simulink model "non_ACC"  (R2021b)
settings: Solver=ode5  StartTime=0.0  StopTime=90  FixedStep=1/20  RelTol=1e-3
PreLoadFcn:
  | mbxruntime.callbacks.PreLoadFcn(bdroot);
PostLoadFcn:
  | mbxruntime.callbacks.PostLoadFcn(bdroot);
InitFcn:
  | mbxruntime.callbacks.InitFcn(bdroot);
StartFcn:
  | mbxruntime.callbacks.StartFcn(bdroot);
StopFcn:
  | mbxruntime.callbacks.StopFcn(bdroot);
model workspace: external: MAT-File .\kea_demo_0218_cs_hws.mat (data not in the file)
undefined symbols (not defined in the file): DiscIntNeverNeededParam, kea_demo_0218_cs_1d5c9b61e8e009e5, kea_demo_0218_cs_4669f259e7287783, kea_demo_0218_cs_87ee11d7829c0052, kea_demo_0218_cs_Audi_A3_1_Dynamics_Simple_initialPitch, kea_demo_0218_cs_Audi_A3_1_Dynamics_Simple_initialRoll, kea_demo_0218_cs_Audi_A3_1_Dynamics_Simple_initialX, kea_demo_0218_cs_Audi_A3_1_Dynamics_Simple_initialY, kea_demo_0218_cs_Audi_A3_1_Dynamics_Simple_initialYaw, kea_demo_0218_cs_Audi_A3_1_Dynamics_Simple_initialZ, kea_demo_0218_cs_Audi_A3_1_PathFollower_Preview_1_PathUniqueID, kea_demo_0218_cs_Roewe_550_S_Sedan_1_Dynamics_Simple_initialX, kea_demo_0218_cs_Roewe_550_S_Sedan_1_Dynamics_Simple_initialY, kea_demo_0218_cs_Roewe_550_S_Sedan_1_Dynamics_Simple_initialYaw, kea_demo_0218_cs_Roewe_550_S_Sedan_1_Dynamics_Simple_initialZ, mbxruntime, warningInitialVelocity, x0
libraries: simulink x56, simulink_extras x18
(part 6 of 7)

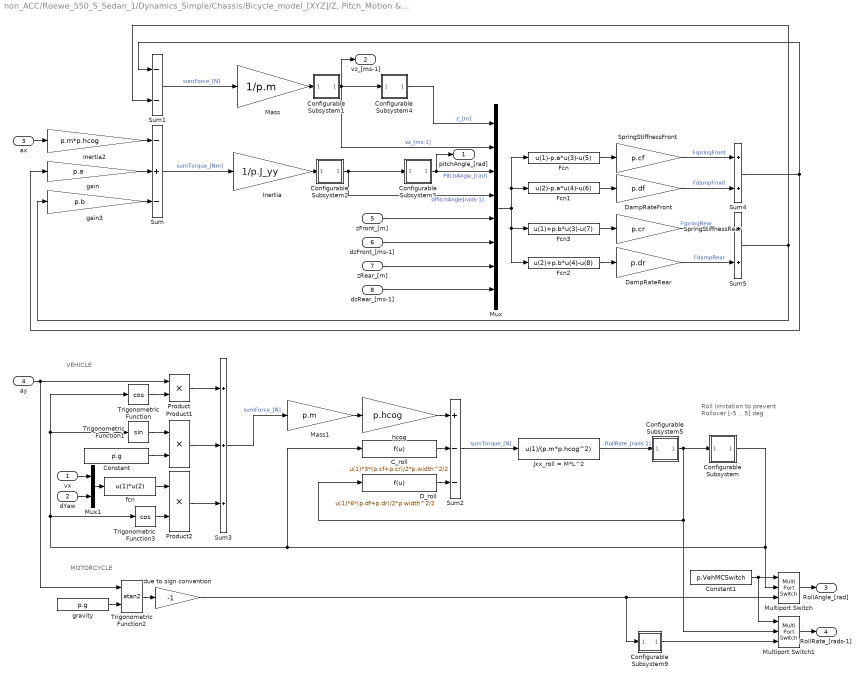
== system non_ACC/Roewe_550_S_Sedan_1/Dynamics_Simple/Chassis/Bicycle_model_[XYZ]/Z, Pitch_Motion & Roll_Motion ==
  note: MOTORCYCLE
  note: VEHICLE
  note: Roll limitation
      | to prevent
      | Rollover
      | [-5 .. 5] deg
  vx : Inport
  dYaw : Inport  Port=2
  ax : Inport  Port=3
  ay : Inport  Port=4
  zFront_[m] : Inport  Port=5
  dzFront_[ms-1] : Inport  Port=6
  zRear_[m] : Inport  Port=7
  dzRear_[ms-1] : Inport  Port=8
  C_roll : Fcn  Expr=u(1)*3*(p.cf+p.cr)/2*p.width^2/2
  Configurable Subsystem : Subsystem  Variant=on  VariantControlMode=label  LabelModeActiveChoice=Continuous  mask{UpperSaturationLimit=+5/180*pi, LowerSaturationLimit=-5/180*pi}
      mask prompts: UpperSaturationLimit "Upper saturation limit"; LowerSaturationLimit "Lower saturation limit"
      mask init: same as non_ACC/Audi_A3_1/Dynamics_Simple/Chassis/Bicycle_model_[XYZ]/Z, Pitch_Motion & Roll_Motion/Configurable Subsystem
      settings: AttributesFormatString=%<BlockChoice>  OpenFcn=BringToFront(gcb);
  Configurable Subsystem1 : Subsystem  Variant=on  VariantControlMode=label  LabelModeActiveChoice=Continuous  mask{IntegrationMethod=Integrator: Forward Euler}
      mask prompts: IntegrationMethod "Integration method"
      mask init: same as non_ACC/Audi_A3_1/Dynamics_Simple/Chassis/MuxDynState/Configurable Subsystem1
      settings: AttributesFormatString=%<BlockChoice>  OpenFcn=BringToFront(gcb);
      mask TypeOptions IntegrationMethod: Integrator: Forward Euler | Integrator: Backward Euler
  Configurable Subsystem2 : Subsystem  Variant=on  VariantControlMode=label  LabelModeActiveChoice=Continuous  mask{IntegrationMethod=Integrator: Forward Euler}
      mask prompts: IntegrationMethod "Integration method"
      mask init: same as non_ACC/Audi_A3_1/Dynamics_Simple/Chassis/MuxDynState/Configurable Subsystem1
      settings: AttributesFormatString=%<BlockChoice>  OpenFcn=BringToFront(gcb);
      mask TypeOptions IntegrationMethod: Integrator: Forward Euler | Integrator: Backward Euler
  Configurable Subsystem3 : Subsystem  Variant=on  VariantControlMode=label  LabelModeActiveChoice=Continuous  mask{IntegrationMethod=Integrator: Forward Euler}
      mask prompts: IntegrationMethod "Integration method"
      mask init: same as non_ACC/Audi_A3_1/Dynamics_Simple/Chassis/MuxDynState/Configurable Subsystem1
      settings: AttributesFormatString=%<BlockChoice>  OpenFcn=BringToFront(gcb);
      mask TypeOptions IntegrationMethod: Integrator: Forward Euler | Integrator: Backward Euler
  Configurable Subsystem4 : Subsystem  Variant=on  VariantControlMode=label  LabelModeActiveChoice=Continuous  mask{IntegrationMethod=Integrator: Forward Euler}
      mask prompts: IntegrationMethod "Integration method"
      mask init: same as non_ACC/Audi_A3_1/Dynamics_Simple/Chassis/MuxDynState/Configurable Subsystem1
      settings: AttributesFormatString=%<BlockChoice>  OpenFcn=BringToFront(gcb);
      mask TypeOptions IntegrationMethod: Integrator: Forward Euler | Integrator: Backward Euler
  Configurable Subsystem5 : Subsystem  Variant=on  VariantControlMode=label  LabelModeActiveChoice=Continuous  mask{IntegrationMethod=Integrator: Forward Euler}
      mask prompts: IntegrationMethod "Integration method"
      mask init: same as non_ACC/Audi_A3_1/Dynamics_Simple/Chassis/MuxDynState/Configurable Subsystem1
      settings: AttributesFormatString=%<BlockChoice>  OpenFcn=BringToFront(gcb);
      mask TypeOptions IntegrationMethod: Integrator: Forward Euler | Integrator: Backward Euler
  Configurable Subsystem9 : Subsystem  Variant=on  VariantControlMode=label  LabelModeActiveChoice=Continuous
      settings: AttributesFormatString=%<BlockChoice>  OpenFcn=BringToFront(gcb);
  Constant : Constant  Value=p.g
  Constant1 : Constant  Value=p.VehMCSwitch
  D_roll : Fcn  Expr=u(1)*6*(p.df+p.dr)/2*p.width^2/2
  DampRateFront : Gain  Gain=p.df  SaturateOnIntegerOverflow=on  OutDataTypeStr=Inherit: Same as input  ParamDataTypeStr=Inherit: Same as input
  DampRateRear : Gain  Gain=p.dr  SaturateOnIntegerOverflow=on  OutDataTypeStr=Inherit: Same as input  ParamDataTypeStr=Inherit: Same as input
  Fcn : Fcn  Expr=u(1)-p.a*u(3)-u(5)
  Fcn1 : Fcn  Expr=u(2)-p.a*u(4)-u(6)
  Fcn2 : Fcn  Expr=u(2)+p.b*u(4)-u(8)
  Fcn3 : Fcn  Expr=u(1)+p.b*u(3)-u(7)
  Inertia : Gain  Gain=1/p.J_yy  SaturateOnIntegerOverflow=on  OutDataTypeStr=Inherit: Same as input  ParamDataTypeStr=Inherit: Same as input
  Inertia2 : Gain  Gain=p.m*p.hcog  SaturateOnIntegerOverflow=on  OutDataTypeStr=Inherit: Same as input  ParamDataTypeStr=Inherit: Same as input
  Jxx_roll = M*L^2 : Fcn  Expr=u(1)/(p.m*p.hcog^2)
  Mass : Gain  Gain=1/p.m  SaturateOnIntegerOverflow=on  OutDataTypeStr=Inherit: Same as input  ParamDataTypeStr=Inherit: Same as input
  Mass1 : Gain  Gain=p.m  SaturateOnIntegerOverflow=on  OutDataTypeStr=Inherit: Same as input  ParamDataTypeStr=Inherit: Same as input
  Multiport Switch : MultiPortSwitch  Inputs=2
  Multiport Switch1 : MultiPortSwitch  Inputs=2
  Mux : Mux  Inputs=8
  Mux1 : Mux  Inputs=2
  Product : Product  RndMeth=Zero
  Product1 : Product  RndMeth=Zero
  Product2 : Product  RndMeth=Zero
  SpringStiffnessFront : Gain  Gain=p.cf  SaturateOnIntegerOverflow=on  OutDataTypeStr=Inherit: Same as input  ParamDataTypeStr=Inherit: Same as input
  SpringStiffnessRear : Gain  Gain=p.cr  SaturateOnIntegerOverflow=on  OutDataTypeStr=Inherit: Same as input  ParamDataTypeStr=Inherit: Same as input
  Sum : Sum  Inputs=-+-  InputSameDT=on  SaturateOnIntegerOverflow=on  OutDataTypeStr=Inherit: Same as first input
  Sum1 : Sum  Inputs=--  InputSameDT=on  SaturateOnIntegerOverflow=on  OutDataTypeStr=Inherit: Same as first input
  Sum2 : Sum  Inputs=+--  InputSameDT=on  SaturateOnIntegerOverflow=on  OutDataTypeStr=Inherit: Same as first input
  Sum3 : Sum  Inputs=+++  InputSameDT=on  SaturateOnIntegerOverflow=on  OutDataTypeStr=Inherit: Same as first input
  Sum4 : Sum  InputSameDT=on  SaturateOnIntegerOverflow=on  OutDataTypeStr=Inherit: Same as first input
  Sum5 : Sum  InputSameDT=on  SaturateOnIntegerOverflow=on  OutDataTypeStr=Inherit: Same as first input
  Trigonometric Function : Trigonometry  Operator=cos
  Trigonometric Function1 : Trigonometry
  Trigonometric Function2 : Trigonometry  Operator=atan2
  Trigonometric Function3 : Trigonometry  Operator=cos
  due to sign convention : Gain  Gain=-1  SaturateOnIntegerOverflow=on  OutDataTypeStr=Inherit: Same as input  ParamDataTypeStr=Inherit: Same as input
  fcn : Fcn  Expr=u(1)*u(2)
  gain : Gain  Gain=p.a  SaturateOnIntegerOverflow=on  OutDataTypeStr=Inherit: Same as input  ParamDataTypeStr=Inherit: Same as input
  gain3 : Gain  Gain=p.b  SaturateOnIntegerOverflow=on  OutDataTypeStr=Inherit: Same as input  ParamDataTypeStr=Inherit: Same as input
  gravity : Constant  Value=p.g
  hcog : Gain  Gain=p.hcog  SaturateOnIntegerOverflow=on  OutDataTypeStr=Inherit: Same as input  ParamDataTypeStr=Inherit: Same as input
  pitchAngle_[rad] : Outport  VectorParamsAs1DForOutWhenUnconnected=off
  vz_[ms-1] : Outport  Port=2  VectorParamsAs1DForOutWhenUnconnected=off
  RollAngle_[rad] : Outport  Port=3  VectorParamsAs1DForOutWhenUnconnected=off
  RollRate_[rads-1] : Outport  Port=4  VectorParamsAs1DForOutWhenUnconnected=off
  wires:
  Inertia/1 -> Configurable Subsystem2/1(In1)
  Configurable Subsystem2/1(Out1) -> Configurable Subsystem3/1(In1), Mux/4  "dPitchAngle[rads-1]"
  Mass/1 -> Configurable Subsystem1/1(In1)
  Configurable Subsystem1/1(Out1) -> Configurable Subsystem4/1(In1), Mux/2, vz_[ms-1]/1  "vz_[ms-1]"
  ax/1 -> Inertia2/1
  Inertia2/1 -> Sum/1
  zFront_[m]/1 -> Mux/5
  dzFront_[ms-1]/1 -> Mux/6
  zRear_[m]/1 -> Mux/7
  dzRear_[ms-1]/1 -> Mux/8
  Configurable Subsystem4/1(Out1) -> Mux/1  "z_[m]"
  SpringStiffnessFront/1 -> Sum4/1  "FspringFront"
  DampRateFront/1 -> Sum4/2  "FdampFront"
  DampRateRear/1 -> Sum5/2  "FdampRear"
  SpringStiffnessRear/1 -> Sum5/1  "FspringRear"
  gain3/1 -> Sum/3
  gain/1 -> Sum/2
  Configurable Subsystem3/1(Out1) -> Mux/3, pitchAngle_[rad]/1  "PitchAngle_[rad]"
  Sum4/1 -> Sum1/1, gain/1
  Sum5/1 -> gain3/1, Sum1/2
  Sum2/1 -> Jxx_roll = M*L^2/1  "sumTorque_[N]"
  Jxx_roll = M*L^2/1 -> Configurable Subsystem5/1(In1)  "RollRate_[rads-2]"
  Configurable Subsystem5/1(Out1) -> Configurable Subsystem/1(In1), D_roll/1, Multiport Switch1/2
  Configurable Subsystem/1(Out1) -> C_roll/1, Trigonometric Function1/1, Trigonometric Function/1, Trigonometric Function3/1, Multiport Switch/2
  Trigonometric Function/1 -> Product/2
  ay/1 -> Product/1, Trigonometric Function2/1
  Trigonometric Function1/1 -> Product1/1
  Constant/1 -> Product1/2
  Product/1 -> Sum3/1
  Product1/1 -> Sum3/2
  Mass1/1 -> hcog/1
  hcog/1 -> Sum2/1
  C_roll/1 -> Sum2/2
  D_roll/1 -> Sum2/3
  Mux/1 -> Fcn2/1, Fcn3/1, Fcn/1, Fcn1/1
  Fcn/1 -> SpringStiffnessFront/1
  Fcn1/1 -> DampRateFront/1
  Fcn3/1 -> SpringStiffnessRear/1
  Fcn2/1 -> DampRateRear/1
  due to sign convention/1 -> Configurable Subsystem9/1(In1), Multiport Switch/3
  Trigonometric Function2/1 -> due to sign convention/1
  gravity/1 -> Trigonometric Function2/2
  Constant1/1 -> Multiport Switch/1, Multiport Switch1/1
  Multiport Switch/1 -> RollAngle_[rad]/1
  Multiport Switch1/1 -> RollRate_[rads-1]/1
  Configurable Subsystem9/1(Out1) -> Multiport Switch1/3
  Mux1/1 -> fcn/1
  vx/1 -> Mux1/1
  dYaw/1 -> Mux1/2
  fcn/1 -> Product2/1
  Trigonometric Function3/1 -> Product2/2
  Product2/1 -> Sum3/3
  Sum/1 -> Inertia/1  "sumTorque_[Nm]"
  Sum1/1 -> Mass/1  "sumForce_[N]"
  Sum3/1 -> Mass1/1  "sumForce_[N]"

== system non_ACC/Roewe_550_S_Sedan_1/Dynamics_Simple/Chassis/FrontTyre/AlphaFront ==
  In : Inport
  Abs : Abs
  Compare To Constant : simulink/Logic and Bit Operations/Compare To Constant  relop=>  const=0  OutDataTypeStr=uint8  ZeroCross=off
  Enabled Subsystem : Subsystem  TreatAsAtomicUnit=on
  Selector : Selector  IndexOptions=Index vector (dialog)  Indices=1  OutputSizes=1
  Alpha : Outport  VectorParamsAs1DForOutWhenUnconnected=off
  wires:
  Selector/1 -> Abs/1
  Compare To Constant/1 -> Enabled Subsystem/Enable
  Enabled Subsystem/1(Alpha) -> Alpha/1
  In/1 -> Enabled Subsystem/1(In), Selector/1
  Abs/1 -> Compare To Constant/1

== system non_ACC/Roewe_550_S_Sedan_1/Dynamics_Simple/Chassis/FrontTyre/Configurable Subsystem ==
  In1 : Inport
  In2 : Inport  Port=2
  Discrete-Time Integrator : Subsystem  VariantControl=Discrete
  Integrator : Subsystem  VariantControl=Continuous
  Out1 : Outport  VectorParamsAs1DForOutWhenUnconnected=off

== system non_ACC/Roewe_550_S_Sedan_1/Dynamics_Simple/Chassis/FrontTyre/Configurable Subsystem1 ==
  In1 : Inport
  In2 : Inport  Port=2
  Discrete-Time Integrator : Subsystem  VariantControl=Discrete
  Integrator : Subsystem  VariantControl=Continuous
  Out1 : Outport  VectorParamsAs1DForOutWhenUnconnected=off

== system non_ACC/Roewe_550_S_Sedan_1/Dynamics_Simple/Chassis/FrontTyre/Prevent_instability_at_low_Vx ==
  note: |vx|
  alpha[rad] : Inport
  In : Inport  Port=2
  Divide : Product  Inputs=**
  Lookup Table : Lookup  InputValues="[0    2.5   ]"  Table="[0.01    1]"  LookUpMeth=Interpolation-Use End Values
  Selector : Selector  InputPortWidth=3  IndexOptions=Index vector (dialog)  Indices=[1]  OutputSizes=1
  alpha [rad] : Outport  VectorParamsAs1DForOutWhenUnconnected=off
  wires:
  In/1 -> Selector/1
  Lookup Table/1 -> Divide/2
  Selector/1 -> Lookup Table/1
  alpha[rad]/1 -> Divide/1
  Divide/1 -> alpha [rad]/1

== system non_ACC/Roewe_550_S_Sedan_1/Dynamics_Simple/Chassis/MuxDynState/Configurable Subsystem1 ==
  In1 : Inport
  Discrete-Time Integrator : Subsystem  VariantControl=Discrete
  Integrator : Subsystem  VariantControl=Continuous
  Out1 : Outport  VectorParamsAs1DForOutWhenUnconnected=off

== system non_ACC/Roewe_550_S_Sedan_1/Dynamics_Simple/Chassis/MuxDynState/Transformation_BODY2GLOBAL ==
  Vvector_BODY_[m/s] : Inport
  angles_BODYwrtGLOB_[rad] : Inport  Port=2
  Dot Product : DotProduct  InputSameDT=on  OutDataTypeStr=Inherit: Inherit via internal rule
  Dot Product1 : DotProduct  InputSameDT=on  OutDataTypeStr=Inherit: Inherit via internal rule
  Dot Product2 : DotProduct  InputSameDT=on  OutDataTypeStr=Inherit: Inherit via internal rule
  Fcn10 : Fcn  Expr=cos(u(1))*sin(u(2))*sin(u(3))-sin(u(1))*cos(u(3))
  Fcn11 : Fcn  Expr=cos(u(1))*sin(u(2))*cos(u(3))+sin(u(1))*sin(u(3))
  Fcn12 : Fcn  Expr=sin(u(1))*cos(u(2))
  Fcn13 : Fcn  Expr=sin(u(1))*sin(u(2))*sin(u(3))+cos(u(1))*cos(u(3))
  Fcn14 : Fcn  Expr=sin(u(1))*sin(u(2))*cos(u(3))-cos(u(1))*sin(u(3))
  Fcn15 : Fcn  Expr=-sin(u(2))
  Fcn16 : Fcn  Expr=cos(u(2))*sin(u(3))
  Fcn17 : Fcn  Expr=cos(u(2))*cos(u(3))
  Fcn9 : Fcn  Expr=cos(u(1))*cos(u(2))
  Mux1 : Mux  Inputs=9
  Mux3 : Mux  Inputs=3
  Selector : Selector  InputPortWidth=9  IndexOptions=Index vector (dialog)  Indices=[1 2 3]  OutputSizes=1
  Selector1 : Selector  InputPortWidth=9  IndexOptions=Index vector (dialog)  Indices=[4 5 6]  OutputSizes=1
  Selector2 : Selector  InputPortWidth=9  IndexOptions=Index vector (dialog)  Indices=[7 8 9]  OutputSizes=1
  rot_xyz 2 rot_zyx : Selector  InputPortWidth=3  IndexOptions=Index vector (dialog)  Indices=[3 2 1]  OutputSizes=1
  Vvector_GLOBAL_[m/s] : Outport  VectorParamsAs1DForOutWhenUnconnected=off
  wires:
  Fcn9/1 -> Mux1/1
  Fcn10/1 -> Mux1/2
  Fcn11/1 -> Mux1/3
  Fcn12/1 -> Mux1/4
  Fcn13/1 -> Mux1/5
  Fcn14/1 -> Mux1/6
  Fcn15/1 -> Mux1/7
  Fcn16/1 -> Mux1/8
  Fcn17/1 -> Mux1/9
  Mux1/1 -> Selector/1, Selector1/1, Selector2/1  "RotationMatrix Visu"
  Selector/1 -> Dot Product/2
  Vvector_BODY_[m/s]/1 -> Dot Product2/1, Dot Product1/1, Dot Product/1
  Dot Product/1 -> Mux3/1
  Selector1/1 -> Dot Product1/2
  Selector2/1 -> Dot Product2/2
  Dot Product2/1 -> Mux3/3
  Dot Product1/1 -> Mux3/2
  rot_xyz 2 rot_zyx/1 -> Fcn9/1, Fcn10/1, Fcn11/1, Fcn12/1, Fcn13/1, Fcn14/1, Fcn15/1, Fcn16/1, Fcn17/1
  Mux3/1 -> Vvector_GLOBAL_[m/s]/1
  angles_BODYwrtGLOB_[rad]/1 -> rot_xyz 2 rot_zyx/1

== system non_ACC/Roewe_550_S_Sedan_1/Dynamics_Simple/Chassis/RearTyre/AlphaRear ==
  In : Inport
  Abs : Abs
  Compare To Constant : simulink/Logic and Bit Operations/Compare To Constant  relop=>  const=0  OutDataTypeStr=uint8  ZeroCross=off
  Enabled Subsystem : Subsystem  TreatAsAtomicUnit=on
  Selector : Selector  IndexOptions=Index vector (dialog)  Indices=1  OutputSizes=1
  Alpha : Outport  VectorParamsAs1DForOutWhenUnconnected=off
  wires:
  Selector/1 -> Abs/1
  Compare To Constant/1 -> Enabled Subsystem/Enable
  Enabled Subsystem/1(Alpha) -> Alpha/1
  In/1 -> Enabled Subsystem/1(In), Selector/1
  Abs/1 -> Compare To Constant/1

== system non_ACC/Roewe_550_S_Sedan_1/Dynamics_Simple/Chassis/RearTyre/Configurable Subsystem ==
  In1 : Inport
  In2 : Inport  Port=2
  Discrete-Time Integrator : Subsystem  VariantControl=Discrete
  Integrator : Subsystem  VariantControl=Continuous
  Out1 : Outport  VectorParamsAs1DForOutWhenUnconnected=off

== system non_ACC/Roewe_550_S_Sedan_1/Dynamics_Simple/Chassis/RearTyre/Configurable Subsystem1 ==
  In1 : Inport
  In2 : Inport  Port=2
  Discrete-Time Integrator : Subsystem  VariantControl=Discrete
  Integrator : Subsystem  VariantControl=Continuous
  Out1 : Outport  VectorParamsAs1DForOutWhenUnconnected=off

== system non_ACC/Roewe_550_S_Sedan_1/Dynamics_Simple/Chassis/RearTyre/Prevent_instability_at_low_Vx ==
  note: |vx|
  alpha[rad] : Inport
  In : Inport  Port=2
  Divide : Product  Inputs=**
  Lookup Table : Lookup  InputValues="[0    2.5   ]"  Table="[0.01    1]"  LookUpMeth=Interpolation-Use End Values
  Selector : Selector  InputPortWidth=3  IndexOptions=Index vector (dialog)  Indices=[1]  OutputSizes=1
  alpha [rad] : Outport  VectorParamsAs1DForOutWhenUnconnected=off
  wires:
  In/1 -> Selector/1
  Lookup Table/1 -> Divide/2
  Selector/1 -> Lookup Table/1
  alpha[rad]/1 -> Divide/1
  Divide/1 -> alpha [rad]/1

== system non_ACC/Roewe_550_S_Sedan_1/Dynamics_Simple/Engine/Configurable Subsystem/Discrete Rate Limiter ==
  In1 : Inport
  Discrete Rate Limiter : DiscreteTransferFcn  Numerator="[  1-exp(-( (TimeStep) / 0.1) )  ]"  Denominator="[  1   -exp(-( (TimeStep) / 0.1) )   ]"  SampleTime=TimeStep
  Out1 : Outport  VectorParamsAs1DForOutWhenUnconnected=off
  wires:
  Discrete Rate Limiter/1 -> Out1/1
  In1/1 -> Discrete Rate Limiter/1

== system non_ACC/Roewe_550_S_Sedan_1/Dynamics_Simple/Engine/Configurable Subsystem/Rate Limiter ==
  In1 : Inport
  Rate Limiter : TransferFcn  Denominator=[0.1 1]
  Out1 : Outport  VectorParamsAs1DForOutWhenUnconnected=off
  wires:
  Rate Limiter/1 -> Out1/1
  In1/1 -> Rate Limiter/1

== system non_ACC/Roewe_550_S_Sedan_1/Dynamics_Simple/Engine/Configurable Subsystem1/Discrete-Time Integrator ==
  In1 : Inport
  Discrete-Time Integrator : DiscreteIntegrator  InitialCondition=p.rot_ini  SampleTime=TimeStep  LimitOutput=on  UpperSaturationLimit=p.rot_upp  LowerSaturationLimit=p.rot_low  ICPrevOutput=DiscIntNeverNeededParam  ICPrevScaledInput=DiscIntNeverNeededParam
  Out1 : Outport  VectorParamsAs1DForOutWhenUnconnected=off
  wires:
  Discrete-Time Integrator/1 -> Out1/1
  In1/1 -> Discrete-Time Integrator/1

== system non_ACC/Roewe_550_S_Sedan_1/Dynamics_Simple/Engine/Configurable Subsystem1/Integrator ==
  In1 : Inport
  Integrator : Integrator  InitialCondition=p.rot_ini  LimitOutput=on  UpperSaturationLimit=p.rot_upp  LowerSaturationLimit=p.rot_low
  Out1 : Outport  VectorParamsAs1DForOutWhenUnconnected=off
  wires:
  Integrator/1 -> Out1/1
  In1/1 -> Integrator/1

== system non_ACC/Roewe_550_S_Sedan_1/Dynamics_Simple/ShiftLogic/Detect Increase/If V0 higher of the from 2->3 shifting velocity ==
  In1 : Inport
  Action Port : ActionPort  PropagateVarSize=During execution  ActionPortLabel="if(u1==1 &  u2==1)"
  Out1 : Outport  VectorParamsAs1DForOutWhenUnconnected=off
  wires:
  In1/1 -> Out1/1

== system non_ACC/Roewe_550_S_Sedan_1/Dynamics_Simple/ShiftLogic/Detect Increase/Other ==
  In1 : Inport
  Action Port : ActionPort  PropagateVarSize=During execution  ActionPortLabel=else
  Data Type Conversion : DataTypeConversion  OutDataTypeStr=double
  Detect Increase : simulink/Logic and Bit Operations/Detect Increase  vinit=0.0  OutDataTypeStr=uint8
  Out1 : Outport  VectorParamsAs1DForOutWhenUnconnected=off
  wires:
  In1/1 -> Detect Increase/1
  Detect Increase/1 -> Data Type Conversion/1
  Data Type Conversion/1 -> Out1/1

== system non_ACC/Roewe_550_S_Sedan_1/Dynamics_Simple/State2Bus1/state2FullState/Transformation_BODY2GLOBAL ==
  Vvector_BODY_[m/s] : Inport
  angles_BODYwrtGLOB_[rad] : Inport  Port=2
  Dot Product : DotProduct  InputSameDT=on  OutDataTypeStr=Inherit: Inherit via internal rule
  Dot Product1 : DotProduct  InputSameDT=on  OutDataTypeStr=Inherit: Inherit via internal rule
  Dot Product2 : DotProduct  InputSameDT=on  OutDataTypeStr=Inherit: Inherit via internal rule
  Fcn10 : Fcn  Expr=cos(u(1))*sin(u(2))*sin(u(3))-sin(u(1))*cos(u(3))
  Fcn11 : Fcn  Expr=cos(u(1))*sin(u(2))*cos(u(3))+sin(u(1))*sin(u(3))
  Fcn12 : Fcn  Expr=sin(u(1))*cos(u(2))
  Fcn13 : Fcn  Expr=sin(u(1))*sin(u(2))*sin(u(3))+cos(u(1))*cos(u(3))
  Fcn14 : Fcn  Expr=sin(u(1))*sin(u(2))*cos(u(3))-cos(u(1))*sin(u(3))
  Fcn15 : Fcn  Expr=-sin(u(2))
  Fcn16 : Fcn  Expr=cos(u(2))*sin(u(3))
  Fcn17 : Fcn  Expr=cos(u(2))*cos(u(3))
  Fcn9 : Fcn  Expr=cos(u(1))*cos(u(2))
  Mux1 : Mux  Inputs=9
  Mux3 : Mux  Inputs=3
  Selector : Selector  InputPortWidth=9  IndexOptions=Index vector (dialog)  Indices=[1 2 3]  OutputSizes=1
  Selector1 : Selector  InputPortWidth=9  IndexOptions=Index vector (dialog)  Indices=[4 5 6]  OutputSizes=1
  Selector2 : Selector  InputPortWidth=9  IndexOptions=Index vector (dialog)  Indices=[7 8 9]  OutputSizes=1
  rot_xyz 2 rot_zyx : Selector  InputPortWidth=3  IndexOptions=Index vector (dialog)  Indices=[3 2 1]  OutputSizes=1
  Vvector_GLOBAL_[m/s] : Outport  VectorParamsAs1DForOutWhenUnconnected=off
  wires:
  angles_BODYwrtGLOB_[rad]/1 -> rot_xyz 2 rot_zyx/1
  Mux3/1 -> Vvector_GLOBAL_[m/s]/1
  rot_xyz 2 rot_zyx/1 -> Fcn17/1, Fcn16/1, Fcn15/1, Fcn14/1, Fcn13/1, Fcn12/1, Fcn11/1, Fcn10/1, Fcn9/1
  Dot Product1/1 -> Mux3/2
  Dot Product2/1 -> Mux3/3
  Selector2/1 -> Dot Product2/2
  Selector1/1 -> Dot Product1/2
  Dot Product/1 -> Mux3/1
  Vvector_BODY_[m/s]/1 -> Dot Product/1, Dot Product1/1, Dot Product2/1
  Selector/1 -> Dot Product/2
  Mux1/1 -> Selector2/1, Selector1/1, Selector/1  "RotationMatrix Visu"
  Fcn17/1 -> Mux1/9
  Fcn16/1 -> Mux1/8
  Fcn15/1 -> Mux1/7
  Fcn14/1 -> Mux1/6
  Fcn13/1 -> Mux1/5
  Fcn12/1 -> Mux1/4
  Fcn11/1 -> Mux1/3
  Fcn10/1 -> Mux1/2
  Fcn9/1 -> Mux1/1

== system non_ACC/Roewe_550_S_Sedan_1/Dynamics_Simple/State2Bus1/state2FullState/Transformation_BODY2GLOBAL1 ==
  POSvector_BODY_[m] : Inport
  angles_BODYwrtGLOB_[rad] : Inport  Port=2
  Dot Product : DotProduct  InputSameDT=on  OutDataTypeStr=Inherit: Inherit via internal rule
  Dot Product1 : DotProduct  InputSameDT=on  OutDataTypeStr=Inherit: Inherit via internal rule
  Dot Product2 : DotProduct  InputSameDT=on  OutDataTypeStr=Inherit: Inherit via internal rule
  Fcn10 : Fcn  Expr=cos(u(1))*sin(u(2))*sin(u(3))-sin(u(1))*cos(u(3))
  Fcn11 : Fcn  Expr=cos(u(1))*sin(u(2))*cos(u(3))+sin(u(1))*sin(u(3))
  Fcn12 : Fcn  Expr=sin(u(1))*cos(u(2))
  Fcn13 : Fcn  Expr=sin(u(1))*sin(u(2))*sin(u(3))+cos(u(1))*cos(u(3))
  Fcn14 : Fcn  Expr=sin(u(1))*sin(u(2))*cos(u(3))-cos(u(1))*sin(u(3))
  Fcn15 : Fcn  Expr=-sin(u(2))
  Fcn16 : Fcn  Expr=cos(u(2))*sin(u(3))
  Fcn17 : Fcn  Expr=cos(u(2))*cos(u(3))
  Fcn9 : Fcn  Expr=cos(u(1))*cos(u(2))
  Mux1 : Mux  Inputs=9
  Mux3 : Mux  Inputs=3
  Selector : Selector  InputPortWidth=9  IndexOptions=Index vector (dialog)  Indices=[1 2 3]  OutputSizes=1
  Selector1 : Selector  InputPortWidth=9  IndexOptions=Index vector (dialog)  Indices=[4 5 6]  OutputSizes=1
  Selector2 : Selector  InputPortWidth=9  IndexOptions=Index vector (dialog)  Indices=[7 8 9]  OutputSizes=1
  rot_xyz 2 rot_zyx : Selector  InputPortWidth=3  IndexOptions=Index vector (dialog)  Indices=[3 2 1]  OutputSizes=1
  POSvector_GLOBAL_[m] : Outport  VectorParamsAs1DForOutWhenUnconnected=off
  wires:
  Fcn9/1 -> Mux1/1
  Fcn10/1 -> Mux1/2
  Fcn11/1 -> Mux1/3
  Fcn12/1 -> Mux1/4
  Fcn13/1 -> Mux1/5
  Fcn14/1 -> Mux1/6
  Fcn15/1 -> Mux1/7
  Fcn16/1 -> Mux1/8
  Fcn17/1 -> Mux1/9
  Mux1/1 -> Selector/1, Selector1/1, Selector2/1  "RotationMatrix"
  Selector/1 -> Dot Product/2
  POSvector_BODY_[m]/1 -> Dot Product2/1, Dot Product1/1, Dot Product/1
  Dot Product/1 -> Mux3/1
  Selector1/1 -> Dot Product1/2
  Selector2/1 -> Dot Product2/2
  Dot Product2/1 -> Mux3/3
  Dot Product1/1 -> Mux3/2
  rot_xyz 2 rot_zyx/1 -> Fcn9/1, Fcn10/1, Fcn11/1, Fcn12/1, Fcn13/1, Fcn14/1, Fcn15/1, Fcn16/1, Fcn17/1
  Mux3/1 -> POSvector_GLOBAL_[m]/1
  angles_BODYwrtGLOB_[rad]/1 -> rot_xyz 2 rot_zyx/1

== system non_ACC/Roewe_550_S_Sedan_1/Dynamics_Simple/State2Bus1/state2FullState/limit roll ==
  RPY : Inport
  Demux : Demux  Outputs=3
  Mux1 : Mux  Inputs=3
  Substitute 90 & 270 deg (and its plurals) : Subsystem
  RPYcor : Outport  VectorParamsAs1DForOutWhenUnconnected=off
  wires:
  Substitute 90 & 270 deg (and its plurals)/1(Subst Angle [rad]) -> Mux1/1
  Mux1/1 -> RPYcor/1
  RPY/1 -> Demux/1
  Demux/3 -> Mux1/3
  Demux/2 -> Mux1/2
  Demux/1 -> Substitute 90 & 270 deg (and its plurals)/1(Angle [rad])

== system non_ACC/Roewe_550_S_Sedan_1/Dynamics_Simple/Transmission/Transmission_Ratio/If Action Neutral ==
  In1 : Inport
  Action Port : ActionPort  InitializeStates=reset  PropagateVarSize=During execution  ActionPortLabel=if(u1 == 0)
  Out1 : Outport  VectorParamsAs1DForOutWhenUnconnected=off
  wires:
  In1/1 -> Out1/1

== system non_ACC/Roewe_550_S_Sedan_1/Dynamics_Simple/Transmission/Transmission_Ratio/If Action Normal ==
  In1 : Inport
  Action Port : ActionPort  InitializeStates=reset  PropagateVarSize=During execution  ActionPortLabel=else
  Out1 : Outport  VectorParamsAs1DForOutWhenUnconnected=off
  wires:
  In1/1 -> Out1/1

== system non_ACC/Roewe_550_S_Sedan_1/Dynamics_Simple/Transmission/Transmission_Ratio/If Action Reverse ==
  In1 : Inport
  Action Port : ActionPort  InitializeStates=reset  PropagateVarSize=During execution  ActionPortLabel=elseif(u1 == -1)
  Reverse : Gain  Gain=-1
  Out1 : Outport  VectorParamsAs1DForOutWhenUnconnected=off
  wires:
  Reverse/1 -> Out1/1
  In1/1 -> Reverse/1

== system non_ACC/Roewe_550_S_Sedan_1/PathFollower_Preview_1/LateralController/SteeringWheelAngle/FirstOrderDynamics ==
  In : Inport
  TimeConstant[s] : Inport  Port=2
  Reset : Inport  Port=3
  x0 : Inport  Port=4
  1|TimeConstant : Product  Inputs=*/  InputSameDT=on  SaturateOnIntegerOverflow=on  OutDataTypeStr=Inherit: Same as first input
  Discrete-Time Integrator : DiscreteIntegrator  ExternalReset=rising  InitialConditionSource=external  InitialCondition=x0  SampleTime=CSSampleTime  ICPrevOutput=DiscIntNeverNeededParam  ICPrevScaledInput=DiscIntNeverNeededParam
  IC : InitialCondition  Value=0
  Saturation : Saturate  UpperLimit=1e300  LowerLimit=0.001
  Sum : Sum  Inputs=-+|  InputSameDT=on  SaturateOnIntegerOverflow=on  OutDataTypeStr=Inherit: Same as first input
  Out : Outport  VectorParamsAs1DForOutWhenUnconnected=off
  wires:
  IC/1 -> Discrete-Time Integrator/3
  In/1 -> Sum/2
  x0/1 -> IC/1
  Reset/1 -> Discrete-Time Integrator/2
  1|TimeConstant/1 -> Discrete-Time Integrator/1
  Sum/1 -> 1|TimeConstant/1
  Saturation/1 -> 1|TimeConstant/2
  TimeConstant[s]/1 -> Saturation/1
  Discrete-Time Integrator/1 -> Out/1, Sum/1

== system non_ACC/Roewe_550_S_Sedan_1/PathFollower_Preview_1/LateralController/SteeringWheelAngle/Sat_Total ==
  In : Inport
  Sat_Limit : Inport  Port=2
  Gain1 : Gain  Gain=-1  SaturateOnIntegerOverflow=on  OutDataTypeStr=Inherit: Same as input  ParamDataTypeStr=Inherit: Same as input
  RelOp_UL : RelationalOperator  RndMeth=Nearest
  RelOp_UL1 : RelationalOperator  Operator=<=  RndMeth=Nearest
  Sum : Sum  Inputs=++|  SaturateOnIntegerOverflow=on
  Switch : Switch  Threshold=0.5  SaturateOnIntegerOverflow=on
  Switch1 : Switch  Threshold=0.5  SaturateOnIntegerOverflow=on
  Sat_Total : Outport  VectorParamsAs1DForOutWhenUnconnected=off
  Sat_Info : Outport  Port=2  VectorParamsAs1DForOutWhenUnconnected=off
  wires:
  Sat_Limit/1 -> Gain1/1, Switch/1, RelOp_UL/2
  RelOp_UL/1 -> Switch/2, Sum/2
  Switch/1 -> RelOp_UL1/1, Switch1/3
  Gain1/1 -> RelOp_UL1/2, Switch1/1
  RelOp_UL1/1 -> Switch1/2, Sum/1
  In/1 -> Switch/3, RelOp_UL/1
  Switch1/1 -> Sat_Total/1
  Sum/1 -> Sat_Info/1

== system non_ACC/Roewe_550_S_Sedan_1/PathFollower_Preview_1/LongitudinalController/If Desired Velocity ~= 0/PID_AWU ==
  e : Inport
  Derivative Gain : Gain  Gain=D  SaturateOnIntegerOverflow=on  OutDataTypeStr=Inherit: Same as input  ParamDataTypeStr=Inherit: Same as input
  Discrete-Time Integrator : DiscreteIntegrator  gainval=1  SampleTime=CSSampleTime  UpperSaturationLimit=100  LowerSaturationLimit=-100  ICPrevOutput=DiscIntNeverNeededParam  ICPrevScaledInput=DiscIntNeverNeededParam
  Filter : DiscreteIntegrator  gainval=1  SampleTime=CSSampleTime  ICPrevOutput=DiscIntNeverNeededParam  ICPrevScaledInput=DiscIntNeverNeededParam
  Integral Gain : Gain  Gain=I  SaturateOnIntegerOverflow=on  OutDataTypeStr=Inherit: Same as input  ParamDataTypeStr=Inherit: Same as input
  Integral Gain1 : Gain  Gain=LongCtrl_AWU  SaturateOnIntegerOverflow=on  OutDataTypeStr=Inherit: Same as input  ParamDataTypeStr=Inherit: Same as input
  Proportional Gain : Gain  Gain=P  SaturateOnIntegerOverflow=on  OutDataTypeStr=Inherit: Same as input  ParamDataTypeStr=Inherit: Same as input
  Saturation : Saturate  UpperLimit=100  LowerLimit=-100
  Sum : Sum  Inputs=+++  InputSameDT=on  SaturateOnIntegerOverflow=on  OutDataTypeStr=Inherit: Same as first input
  Sum1 : Sum  Inputs=|+-  InputSameDT=on  SaturateOnIntegerOverflow=on  OutDataTypeStr=Inherit: Same as first input
  Sum2 : Sum  Inputs=|++  InputSameDT=on  SaturateOnIntegerOverflow=on  OutDataTypeStr=Inherit: Same as first input
  Sum3 : Sum  Inputs=-+|  InputSameDT=on  SaturateOnIntegerOverflow=on  OutDataTypeStr=Inherit: Same as first input
  u : Outport  InitialOutput=0  VectorParamsAs1DForOutWhenUnconnected=off
  wires:
  Integral Gain1/1 -> Sum2/2
  Sum3/1 -> Integral Gain1/1
  Saturation/1 -> Sum3/2, u/1
  Sum2/1 -> Discrete-Time Integrator/1
  Sum1/1 -> Sum/3, Filter/1
  Filter/1 -> Sum1/2
  Derivative Gain/1 -> Sum1/1
  Sum/1 -> Sum3/1, Saturation/1
  e/1 -> Integral Gain/1, Proportional Gain/1, Derivative Gain/1
  Discrete-Time Integrator/1 -> Sum/2
  Proportional Gain/1 -> Sum/1
  Integral Gain/1 -> Sum2/1

== system non_ACC/Audi_A3_1/Dynamics_Simple/Chassis/Bicycle_model_[XYZ]/X_Motion/Air&RoadResistance ==
  vx_[ms-1] : Inport
  Gain : Gain  Gain=1/p.Rw
  Road & Aerodyn Resistances : Fcn  Expr=p.Rroad + p.Rair*u^2
  Saturation1 : Saturate  UpperLimit=5/15  LowerLimit=-5/15
  Sign : Signum
  "[ms-1] 2 [rads-1]" : Gain  Gain=1/p.Rw  SaturateOnIntegerOverflow=on  OutDataTypeStr=Inherit: Same as input  ParamDataTypeStr=Inherit: Same as input
  signed load1 : Product  InputSameDT=on  SaturateOnIntegerOverflow=on  OutDataTypeStr=Inherit: Same as first input
  Resistance_Force : Outport  VectorParamsAs1DForOutWhenUnconnected=off
  wires:
  signed load1/1 -> Resistance_Force/1  "F_[N]"
  vx_[ms-1]/1 -> Road & Aerodyn Resistances/1, "[ms-1] 2 [rads-1]"/1
  Saturation1/1 -> Sign/1
  "[ms-1] 2 [rads-1]"/1 -> Saturation1/1
  Road & Aerodyn Resistances/1 -> Gain/1  "ResistanceTorque_[Nm]"
  Sign/1 -> signed load1/2  "sign"
  Gain/1 -> signed load1/1  "Resistance Force_[N]"

== system non_ACC/Audi_A3_1/Dynamics_Simple/Chassis/Bicycle_model_[XYZ]/X_Motion/BrakeSystem ==
  vx_[ms-1] : Inport
  BrakePressure_[bar] : Inport  Port=2
  Gain : Gain  Gain=1/p.Rw
  Saturation : Saturate  UpperLimit=p.PBrakeMax  LowerLimit=0
  Saturation1 : Saturate  UpperLimit=5/15  LowerLimit=-5/15
  Sign : Signum
  "[ms-1] 2 [rads-1]" : Gain  Gain=1/p.Rw  SaturateOnIntegerOverflow=on  OutDataTypeStr=Inherit: Same as input  ParamDataTypeStr=Inherit: Same as input
  braking Q factor : Gain  Gain=p.Qfac  SaturateOnIntegerOverflow=on  OutDataTypeStr=Inherit: Same as input  ParamDataTypeStr=Inherit: Same as input
  signed load1 : Product  InputSameDT=on  SaturateOnIntegerOverflow=on  OutDataTypeStr=Inherit: Same as first input
  BrakeForce : Outport  VectorParamsAs1DForOutWhenUnconnected=off
  BrakeTorqueAbs : Outport  Port=2  VectorParamsAs1DForOutWhenUnconnected=off
  wires:
  braking Q factor/1 -> BrakeTorqueAbs/1, Gain/1
  BrakePressure_[bar]/1 -> Saturation/1
  Saturation/1 -> braking Q factor/1
  vx_[ms-1]/1 -> "[ms-1] 2 [rads-1]"/1
  Saturation1/1 -> Sign/1
  "[ms-1] 2 [rads-1]"/1 -> Saturation1/1
  Sign/1 -> signed load1/2  "sign"
  signed load1/1 -> BrakeForce/1
  Gain/1 -> signed load1/1

== system non_ACC/Audi_A3_1/Dynamics_Simple/Chassis/Bicycle_model_[XYZ]/X_Motion/Configurable Subsystem ==
  In1 : Inport
  In2 : Inport  Port=2
  In3 : Inport  Port=3
  Discrete-Time Integrator : Subsystem  VariantControl=Discrete
  Integrator : Subsystem  VariantControl=Continuous
  Out1 : Outport  VectorParamsAs1DForOutWhenUnconnected=off

== system non_ACC/Audi_A3_1/Dynamics_Simple/Chassis/Bicycle_model_[XYZ]/X_Motion/Configurable Subsystem1 ==
  In1 : Inport
  Discrete Torsional damping : Subsystem  VariantControl=Discrete
  Torsional damping : Subsystem  VariantControl=Continuous
  Out1 : Outport  VectorParamsAs1DForOutWhenUnconnected=off

== system non_ACC/Audi_A3_1/Dynamics_Simple/Chassis/Bicycle_model_[XYZ]/X_Motion/Max RPM and zero- velocity detection ==
  note: Set to zero after infinite small time-step
  note: Zero velocity detection
  ax : Inport
  Drive Torque : Inport  Port=2
  Brake Torque : Inport  Port=3
  v0 : Inport  Port=4
  vx : Inport  Port=5
  Abs : Abs
  Abs1 : Abs
  Compare To Zero : simulink/Logic and Bit Operations/Compare To Zero  relop=<=  OutDataTypeStr=boolean  ZeroCross=off
  Compare To Zero1 : simulink/Logic and Bit Operations/Compare To Zero  relop=>=  OutDataTypeStr=boolean  ZeroCross=off
  Compare To Zero2 : simulink/Logic and Bit Operations/Compare To Zero  relop=>=  OutDataTypeStr=boolean  ZeroCross=off
  Compare To Zero3 : simulink/Logic and Bit Operations/Compare To Zero  relop=<=  OutDataTypeStr=boolean  ZeroCross=off
  Configurable Subsystem : Subsystem  Variant=on  VariantControlMode=label  LabelModeActiveChoice=Continuous
      settings: AttributesFormatString=%<BlockChoice>  OpenFcn=BringToFront(gcb);
  Constant : Constant
  Constant1 : Constant
  Logical Operator : Logic  AllPortsSameDT=off  OutDataTypeStr=boolean
  Logical Operator1 : Logic  AllPortsSameDT=off  OutDataTypeStr=boolean
  Logical Operator2 : Logic  Operator=NOT  AllPortsSameDT=off  OutDataTypeStr=boolean
  Logical Operator3 : Logic  AllPortsSameDT=off  OutDataTypeStr=boolean
  Logical Operator4 : Logic  Operator=OR  AllPortsSameDT=off  OutDataTypeStr=boolean
  Memory : Memory
  Memory1 : Memory
  Memory2 : Memory
  Product : Product  RndMeth=Zero
  Relational Operator : RelationalOperator  Operator=<  OutDataTypeStr=boolean  RndMeth=Nearest
  SR-Memory : Subsystem
  Sum : Sum  Inputs=|-+
  Switch : Switch  Criteria=u2 ~= 0  Threshold=0.5
  ax is 0 : Constant  Value=0
  ax_out : Outport  VectorParamsAs1DForOutWhenUnconnected=off
  vx_reset : Outport  Port=2  VectorParamsAs1DForOutWhenUnconnected=off
  x0 : Outport  Port=3  VectorParamsAs1DForOutWhenUnconnected=off
  wires:
  Logical Operator4/1 -> Logical Operator1/1
  vx/1 -> Compare To Zero/1, Compare To Zero2/1, Memory2/1, Memory/1  "vx"
  Memory2/1 -> Compare To Zero3/1
  Compare To Zero2/1 -> Logical Operator3/1
  Compare To Zero3/1 -> Logical Operator3/2
  Logical Operator3/1 -> Logical Operator4/2  "zero-crossing backward"
  Memory/1 -> Compare To Zero1/1
  Compare To Zero/1 -> Logical Operator/1
  Compare To Zero1/1 -> Logical Operator/2
  Logical Operator/1 -> Logical Operator4/1  "zero-crossing forward"
  Abs/1 -> Relational Operator/1
  Abs1/1 -> Relational Operator/2
  Drive Torque/1 -> Abs/1
  Brake Torque/1 -> Abs1/1
  Relational Operator/1 -> Logical Operator1/2, Logical Operator2/1
  Logical Operator1/1 -> SR-Memory/2(Set)
  Constant/1 -> SR-Memory/1(Signal)
  Logical Operator2/1 -> SR-Memory/3(Reset)
  SR-Memory/1(Out) -> Sum/1, Memory1/1
  Switch/1 -> ax_out/1
  Sum/1 -> Switch/2
  ax is 0/1 -> Switch/3
  Constant1/1 -> Sum/2
  v0/1 -> Product/1
  Product/1 -> x0/1
  Configurable Subsystem/1(Out1) -> Product/2
  ax/1 -> Switch/1  "ax"
  Memory1/1 -> vx_reset/1  "vx"

== system non_ACC/Audi_A3_1/Dynamics_Simple/Chassis/Bicycle_model_[XYZ]/Y & Yaw_Motion/Configurable Subsystem ==
  In1 : Inport
  In2 : Inport  Port=2
  Discrete-Time Integrator : Subsystem  VariantControl=Discrete
  Integrator : Subsystem  VariantControl=Continuous
  Out1 : Outport  VectorParamsAs1DForOutWhenUnconnected=off

== system non_ACC/Audi_A3_1/Dynamics_Simple/Chassis/Bicycle_model_[XYZ]/Y & Yaw_Motion/Configurable Subsystem1 ==
  In1 : Inport
  Discrete-Time Integrator : Subsystem  VariantControl=Discrete
  Integrator : Subsystem  VariantControl=Continuous
  Out1 : Outport  VectorParamsAs1DForOutWhenUnconnected=off

== system non_ACC/Audi_A3_1/Dynamics_Simple/Chassis/Bicycle_model_[XYZ]/Y & Yaw_Motion/Configurable Subsystem2 ==
  In1 : Inport
  In2 : Inport  Port=2
  Discrete-Time Integrator : Subsystem  VariantControl=Discrete
  Integrator : Subsystem  VariantControl=Continuous
  Out1 : Outport  VectorParamsAs1DForOutWhenUnconnected=off

== system non_ACC/Audi_A3_1/Dynamics_Simple/Chassis/Bicycle_model_[XYZ]/Z, Pitch_Motion & Roll_Motion/Configurable Subsystem ==
  In1 : Inport
  Discrete-Time Integrator : Subsystem  VariantControl=Discrete
  Integrator : Subsystem  VariantControl=Continuous
  Out1 : Outport  VectorParamsAs1DForOutWhenUnconnected=off

== system non_ACC/Audi_A3_1/Dynamics_Simple/Chassis/Bicycle_model_[XYZ]/Z, Pitch_Motion & Roll_Motion/Configurable Subsystem1 ==
  In1 : Inport
  Discrete-Time Integrator : Subsystem  VariantControl=Discrete
  Integrator : Subsystem  VariantControl=Continuous
  Out1 : Outport  VectorParamsAs1DForOutWhenUnconnected=off

== system non_ACC/Audi_A3_1/Dynamics_Simple/Chassis/Bicycle_model_[XYZ]/Z, Pitch_Motion & Roll_Motion/Configurable Subsystem2 ==
  In1 : Inport
  Discrete-Time Integrator : Subsystem  VariantControl=Discrete
  Integrator : Subsystem  VariantControl=Continuous
  Out1 : Outport  VectorParamsAs1DForOutWhenUnconnected=off

== system non_ACC/Audi_A3_1/Dynamics_Simple/Chassis/Bicycle_model_[XYZ]/Z, Pitch_Motion & Roll_Motion/Configurable Subsystem3 ==
  In1 : Inport
  Discrete-Time Integrator : Subsystem  VariantControl=Discrete
  Integrator : Subsystem  VariantControl=Continuous
  Out1 : Outport  VectorParamsAs1DForOutWhenUnconnected=off

== system non_ACC/Audi_A3_1/Dynamics_Simple/Chassis/Bicycle_model_[XYZ]/Z, Pitch_Motion & Roll_Motion/Configurable Subsystem4 ==
  In1 : Inport
  Discrete-Time Integrator : Subsystem  VariantControl=Discrete
  Integrator : Subsystem  VariantControl=Continuous
  Out1 : Outport  VectorParamsAs1DForOutWhenUnconnected=off

== system non_ACC/Audi_A3_1/Dynamics_Simple/Chassis/Bicycle_model_[XYZ]/Z, Pitch_Motion & Roll_Motion/Configurable Subsystem5 ==
  In1 : Inport
  Discrete-Time Integrator : Subsystem  VariantControl=Discrete
  Integrator : Subsystem  VariantControl=Continuous
  Out1 : Outport  VectorParamsAs1DForOutWhenUnconnected=off

== system non_ACC/Audi_A3_1/Dynamics_Simple/Chassis/Bicycle_model_[XYZ]/Z, Pitch_Motion & Roll_Motion/Configurable Subsystem9 ==
  In1 : Inport
  Derivative : Subsystem  VariantControl=Continuous
  Discrete Derivative : Subsystem  VariantControl=Discrete
      mask Display: dpoly(['k (z-1)'] , ['Ts z'] ,'');
  Out1 : Outport  VectorParamsAs1DForOutWhenUnconnected=off

== system non_ACC/Audi_A3_1/Dynamics_Simple/Chassis/FrontTyre/AlphaFront/Enabled Subsystem ==
  In : Inport
  Enable : EnablePort  PropagateVarSize=During execution
  AlphaFront : Fcn  Expr=-atan( (u(2)+u(3)*p.a)/u(1) )
  Alpha : Outport  OutputWhenDisabled=reset  InitialOutput=[0]  VectorParamsAs1DForOutWhenUnconnected=off
  wires:
  AlphaFront/1 -> Alpha/1
  In/1 -> AlphaFront/1

== system non_ACC/Audi_A3_1/Dynamics_Simple/Chassis/FrontTyre/Configurable Subsystem/Discrete-Time Integrator ==
  In1 : Inport
  In2 : Inport  Port=2
  Discrete-Time Integrator : DiscreteIntegrator  ExternalReset=level  SampleTime=TimeStep  LimitOutput=on  UpperSaturationLimit=1  LowerSaturationLimit=-1  ICPrevOutput=DiscIntNeverNeededParam  ICPrevScaledInput=DiscIntNeverNeededParam
  Out1 : Outport  VectorParamsAs1DForOutWhenUnconnected=off
  wires:
  Discrete-Time Integrator/1 -> Out1/1
  In2/1 -> Discrete-Time Integrator/2
  In1/1 -> Discrete-Time Integrator/1

== system non_ACC/Audi_A3_1/Dynamics_Simple/Chassis/FrontTyre/Configurable Subsystem/Integrator ==
  In1 : Inport
  In2 : Inport  Port=2
  Integrator : Integrator  ExternalReset=level  LimitOutput=on  UpperSaturationLimit=1  LowerSaturationLimit=-1
  Out1 : Outport  VectorParamsAs1DForOutWhenUnconnected=off
  wires:
  Integrator/1 -> Out1/1
  In2/1 -> Integrator/2
  In1/1 -> Integrator/1

== system non_ACC/Audi_A3_1/Dynamics_Simple/Chassis/FrontTyre/Configurable Subsystem1/Discrete-Time Integrator ==
  In1 : Inport
  In2 : Inport  Port=2
  Discrete-Time Integrator : DiscreteIntegrator  ExternalReset=level  SampleTime=TimeStep  ICPrevOutput=DiscIntNeverNeededParam  ICPrevScaledInput=DiscIntNeverNeededParam
  Out1 : Outport  VectorParamsAs1DForOutWhenUnconnected=off
  wires:
  Discrete-Time Integrator/1 -> Out1/1
  In2/1 -> Discrete-Time Integrator/2
  In1/1 -> Discrete-Time Integrator/1

== system non_ACC/Audi_A3_1/Dynamics_Simple/Chassis/FrontTyre/Configurable Subsystem1/Integrator ==
  In1 : Inport
  In2 : Inport  Port=2
  Integrator : Integrator  ExternalReset=level
  Out1 : Outport  VectorParamsAs1DForOutWhenUnconnected=off
  wires:
  Integrator/1 -> Out1/1
  In2/1 -> Integrator/2
  In1/1 -> Integrator/1

== system non_ACC/Audi_A3_1/Dynamics_Simple/Chassis/MuxDynState/Configurable Subsystem1/Discrete-Time Integrator ==
  In1 : Inport
  Discrete-Time Integrator : DiscreteIntegrator  SampleTime=TimeStep  ICPrevOutput=DiscIntNeverNeededParam  ICPrevScaledInput=DiscIntNeverNeededParam
  Out1 : Outport  VectorParamsAs1DForOutWhenUnconnected=off
  wires:
  Discrete-Time Integrator/1 -> Out1/1
  In1/1 -> Discrete-Time Integrator/1

== system non_ACC/Audi_A3_1/Dynamics_Simple/Chassis/MuxDynState/Configurable Subsystem1/Integrator ==
  In1 : Inport
  Integrator : Integrator
  Out1 : Outport  VectorParamsAs1DForOutWhenUnconnected=off
  wires:
  Integrator/1 -> Out1/1
  In1/1 -> Integrator/1

== system non_ACC/Audi_A3_1/Dynamics_Simple/Chassis/RearTyre/AlphaRear/Enabled Subsystem ==
  In : Inport
  Enable : EnablePort  PropagateVarSize=During execution
  AlphaRear : Fcn  Expr=-atan( (u(2)-u(3)*p.b)/u(1) )
  Alpha : Outport  OutputWhenDisabled=reset  InitialOutput=[0]  VectorParamsAs1DForOutWhenUnconnected=off
  wires:
  AlphaRear/1 -> Alpha/1
  In/1 -> AlphaRear/1

== system non_ACC/Audi_A3_1/Dynamics_Simple/Chassis/RearTyre/Configurable Subsystem/Discrete-Time Integrator ==
  In1 : Inport
  In2 : Inport  Port=2
  Discrete-Time Integrator : DiscreteIntegrator  ExternalReset=level  SampleTime=TimeStep  ICPrevOutput=DiscIntNeverNeededParam  ICPrevScaledInput=DiscIntNeverNeededParam
  Out1 : Outport  VectorParamsAs1DForOutWhenUnconnected=off
  wires:
  Discrete-Time Integrator/1 -> Out1/1
  In2/1 -> Discrete-Time Integrator/2
  In1/1 -> Discrete-Time Integrator/1

== system non_ACC/Audi_A3_1/Dynamics_Simple/Chassis/RearTyre/Configurable Subsystem/Integrator ==
  In1 : Inport
  In2 : Inport  Port=2
  Integrator : Integrator  ExternalReset=level
  Out1 : Outport  VectorParamsAs1DForOutWhenUnconnected=off
  wires:
  Integrator/1 -> Out1/1
  In2/1 -> Integrator/2
  In1/1 -> Integrator/1

== system non_ACC/Audi_A3_1/Dynamics_Simple/Chassis/RearTyre/Configurable Subsystem1/Discrete-Time Integrator ==
  In1 : Inport
  In2 : Inport  Port=2
  Discrete-Time Integrator : DiscreteIntegrator  ExternalReset=level  SampleTime=TimeStep  LimitOutput=on  UpperSaturationLimit=1  LowerSaturationLimit=-1  ICPrevOutput=DiscIntNeverNeededParam  ICPrevScaledInput=DiscIntNeverNeededParam
  Out1 : Outport  VectorParamsAs1DForOutWhenUnconnected=off
  wires:
  Discrete-Time Integrator/1 -> Out1/1
  In2/1 -> Discrete-Time Integrator/2
  In1/1 -> Discrete-Time Integrator/1

== system non_ACC/Audi_A3_1/Dynamics_Simple/Chassis/RearTyre/Configurable Subsystem1/Integrator ==
  In1 : Inport
  In2 : Inport  Port=2
  Integrator : Integrator  ExternalReset=level  LimitOutput=on  UpperSaturationLimit=1  LowerSaturationLimit=-1
  Out1 : Outport  VectorParamsAs1DForOutWhenUnconnected=off
  wires:
  Integrator/1 -> Out1/1
  In2/1 -> Integrator/2
  In1/1 -> Integrator/1

== system non_ACC/Audi_A3_1/Dynamics_Simple/State2Bus1/state2FullState/limit roll/Substitute 90 & 270 deg (and its plurals) ==
  Angle [rad] : Inport
  270 deg detection : simulink/Model Verification/Check  Static Gap  Description=u <= 269.5 || 270.5 <= u  max=270.5  max_included=on  min=269.5  min_included=on  enabled=on  stopWhenAssertionFail=off  export=on  icon=graphic
      settings: SourceProductBaseCode=SL
  90 deg detection : simulink/Model Verification/Check  Static Gap  Description=u <= 89.5 || 90.5 <= u  max=90.5  max_included=on  min=89.5  min_included=on  enabled=on  stopWhenAssertionFail=off  export=on  icon=graphic
      settings: SourceProductBaseCode=SL
  Angle -360 to +360 deg limiter : Subsystem
  Degrees to Radians : simulink_extras/Transformations/Degrees to Radians
  Radians to Degrees : simulink_extras/Transformations/Radians to Degrees
  Substitution Value : Constant  Value=269.5
  Substitution Value : Constant  Value=89.5
  Switch : Switch  Threshold=0.5
  Switch1 : Switch  Threshold=0.5
  Subst Angle [rad] : Outport  VectorParamsAs1DForOutWhenUnconnected=off
  wires:
  Angle [rad]/1 -> Radians to Degrees/1
  Degrees to Radians/1 -> Subst Angle [rad]/1
  Radians to Degrees/1 -> Angle -360 to +360 deg limiter/1(Angle [deg])
  Switch1/1 -> Degrees to Radians/1
  Substitution Value/1 -> Switch1/3
  270 deg detection/1 -> Switch1/2
  Switch/1 -> Switch1/1, 270 deg detection/1
  Substitution Value/1 -> Switch/3
  90 deg detection/1 -> Switch/2
  Angle -360 to +360 deg limiter/1(LimAngle [deg]) -> 90 deg detection/1, Switch/1

== system non_ACC/Roewe_550_S_Sedan_1/Dynamics_Simple/Chassis/Bicycle_model_[XYZ]/X_Motion/Air&RoadResistance ==
  vx_[ms-1] : Inport
  Gain : Gain  Gain=1/p.Rw
  Road & Aerodyn Resistances : Fcn  Expr=p.Rroad + p.Rair*u^2
  Saturation1 : Saturate  UpperLimit=5/15  LowerLimit=-5/15
  Sign : Signum
  "[ms-1] 2 [rads-1]" : Gain  Gain=1/p.Rw  SaturateOnIntegerOverflow=on  OutDataTypeStr=Inherit: Same as input  ParamDataTypeStr=Inherit: Same as input
  signed load1 : Product  InputSameDT=on  SaturateOnIntegerOverflow=on  OutDataTypeStr=Inherit: Same as first input
  Resistance_Force : Outport  VectorParamsAs1DForOutWhenUnconnected=off
  wires:
  signed load1/1 -> Resistance_Force/1  "F_[N]"
  vx_[ms-1]/1 -> Road & Aerodyn Resistances/1, "[ms-1] 2 [rads-1]"/1
  Saturation1/1 -> Sign/1
  "[ms-1] 2 [rads-1]"/1 -> Saturation1/1
  Road & Aerodyn Resistances/1 -> Gain/1  "ResistanceTorque_[Nm]"
  Sign/1 -> signed load1/2  "sign"
  Gain/1 -> signed load1/1  "Resistance Force_[N]"

== system non_ACC/Roewe_550_S_Sedan_1/Dynamics_Simple/Chassis/Bicycle_model_[XYZ]/X_Motion/BrakeSystem ==
  vx_[ms-1] : Inport
  BrakePressure_[bar] : Inport  Port=2
  Gain : Gain  Gain=1/p.Rw
  Saturation : Saturate  UpperLimit=p.PBrakeMax  LowerLimit=0
  Saturation1 : Saturate  UpperLimit=5/15  LowerLimit=-5/15
  Sign : Signum
  "[ms-1] 2 [rads-1]" : Gain  Gain=1/p.Rw  SaturateOnIntegerOverflow=on  OutDataTypeStr=Inherit: Same as input  ParamDataTypeStr=Inherit: Same as input
  braking Q factor : Gain  Gain=p.Qfac  SaturateOnIntegerOverflow=on  OutDataTypeStr=Inherit: Same as input  ParamDataTypeStr=Inherit: Same as input
  signed load1 : Product  InputSameDT=on  SaturateOnIntegerOverflow=on  OutDataTypeStr=Inherit: Same as first input
  BrakeForce : Outport  VectorParamsAs1DForOutWhenUnconnected=off
  BrakeTorqueAbs : Outport  Port=2  VectorParamsAs1DForOutWhenUnconnected=off
  wires:
  braking Q factor/1 -> BrakeTorqueAbs/1, Gain/1
  BrakePressure_[bar]/1 -> Saturation/1
  Saturation/1 -> braking Q factor/1
  vx_[ms-1]/1 -> "[ms-1] 2 [rads-1]"/1
  Saturation1/1 -> Sign/1
  "[ms-1] 2 [rads-1]"/1 -> Saturation1/1
  Sign/1 -> signed load1/2  "sign"
  signed load1/1 -> BrakeForce/1
  Gain/1 -> signed load1/1

== system non_ACC/Roewe_550_S_Sedan_1/Dynamics_Simple/Chassis/Bicycle_model_[XYZ]/X_Motion/Configurable Subsystem ==
  In1 : Inport
  In2 : Inport  Port=2
  In3 : Inport  Port=3
  Discrete-Time Integrator : Subsystem  VariantControl=Discrete
  Integrator : Subsystem  VariantControl=Continuous
  Out1 : Outport  VectorParamsAs1DForOutWhenUnconnected=off

== system non_ACC/Roewe_550_S_Sedan_1/Dynamics_Simple/Chassis/Bicycle_model_[XYZ]/X_Motion/Configurable Subsystem1 ==
  In1 : Inport
  Discrete Torsional damping : Subsystem  VariantControl=Discrete
  Torsional damping : Subsystem  VariantControl=Continuous
  Out1 : Outport  VectorParamsAs1DForOutWhenUnconnected=off
